simulink model "HOSTFOCwithLOAD"  (R2024b)
settings: Solver=FixedStepDiscrete  StartTime=0.0  StopTime=inf  RelTol=1e-3  EnableMultiTasking=on
PreLoadFcn:
  | % 打开/运行模型时初始化基工作区变量，避免每次启动都要“更新图”
  | if ~exist('dataType','var')
  |     dataType = 'single';   % Data_Conditioning 变体控制（Float/single，与目标机一致）
  | end
  | if ~exist('Ts','var')
  |     Ts = 5e-05;             % 20 kHz，与目标机一致
  | end
  | if ~exist('CalModeP','var')
  |     CalModeP = Simulink.Parameter(uint16(0));
  |     CalModeP.DataType = 'uint16';
  |     CalModeP.CoderInfo.StorageClass = 'Auto';
  | end
InitFcn:
  | % 打开/运行模型时初始化基工作区变量，避免每次启动都要“更新图”
  | if ~exist('dataType','var')
  |     dataType = 'single';   % Data_Conditioning 变体控制（Float/single，与目标机一致）
  | end
  | if ~exist('Ts','var')
  |     Ts = 5e-05;             % 20 kHz，与目标机一致
  | end
  | if exist('CalModeP','var') && isa(CalModeP,'Simulink.Parameter')
  |     CalModeP.Value = uint16(0);
  | else
  |     CalModeP = Simulink.Parameter(uint16(0));
  |     CalModeP.DataType = 'uint16';
  |     CalModeP.CoderInfo.StorageClass = 'Auto';
  | end
undefined symbols (not defined in the file or in its folder): PU_System_motor1, PU_System_motor2
libraries: instrumentseriallib x6, simulink x3
settings Model: Creator=The MathWorks, Inc.  LastModifiedBy=admin
settings SolverCC: AllowMultiTaskInputOutput=on  AlgebraicLoopSolver=TrustRegion  MaxZcPerStep=1
settings DataIOCC: LimitDataPoints=on  SaveFormat=Array  ReturnWorkspaceOutputs=off
settings OptimizationCC: LifeSpan=1  EfficientTunableParamExpr=on
settings DebuggingCC: UnderspecifiedInitializationDetection=Classic  MergeDetectMultiDrivingBlocksExec=none  SolverPrmCheckMsg=warning  ParameterPrecisionLossMsg=none  UnconnectedInputMsg=warning  UnconnectedOutputMsg=warning  UnconnectedLineMsg=warning  AllowSymbolicDim=off  PregeneratedLibrarySubsystemCodeDiagnostic=none  SFUnexpectedBacktrackingDiag=warning  SFNoUnconditionalDefaultTransitionDiag=warning  SFExecutionAtInitializationDiag=none  ArithmeticOperatorsInVariantConditions=warning
settings HardwareCC: ProdBitPerPointer=32  ProdLargestAtomicFloat=None  ProdIntDivRoundTo=Undefined  ProdEndianess=Unspecified  ProdWordSize=32  ProdHWDeviceType=32-bit Generic
settings ModelReferenceCC: EnableRefExpFcnMdlSchedulingChecks=on  PropagateSignalLabelsOutOfModel=off
settings SFSimCC: SimUseLocalCustomCode=off  MATLABDynamicMemAlloc=off
settings RTWCC: Description=Real-Time Workshop Embedded Coder  SystemTargetFile=ert.tlc  TemplateMakefile=ert_default_tmf  GenerateReport=on  RTWUseLocalCustomCode=off  IncludeHyperlinkInReport=on  LaunchReport=on  GenerateTraceInfo=on  GenerateTraceReport=on  GenerateTraceReportSl=on  GenerateTraceReportSf=on  GenerateTraceReportEml=on  GPUComputeCapability=3.5  DLArmComputeVersion=19.05
settings CodeAppCC: IgnoreCustomStorageClasses=off  StateflowObjectComments=on  InternalIdentifier=Classic
settings ERTTargetCC: MultiwordLength=2048  GenerateSampleERTMain=on  InlinedParameterPlacement=Hierarchical  ERTCustomFileTemplate=example_file_process.tlc  ConvertIfToSwitch=off  SuppressUnreachableDefaultCases=off  DynamicArrayContainerType=coder::array
settings ConfigComp: CovMetricSettings=dw  CovSaveCumulativeToWorkspaceVar=on  CovSaveSingleToWorkspaceVar=on  CovExternalEMLEnable=off  CovSFcnEnable=off

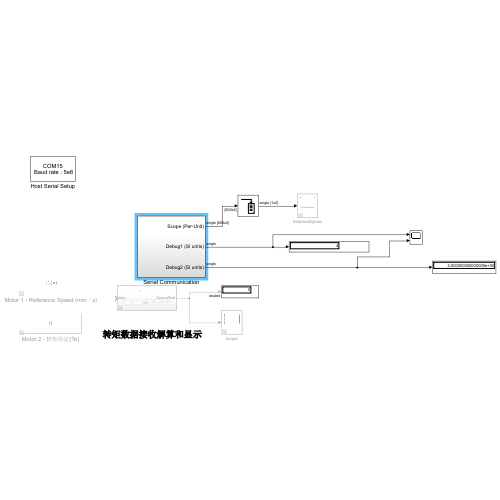
[thumbnail: Simulink's stored preview of the top-level diagram]
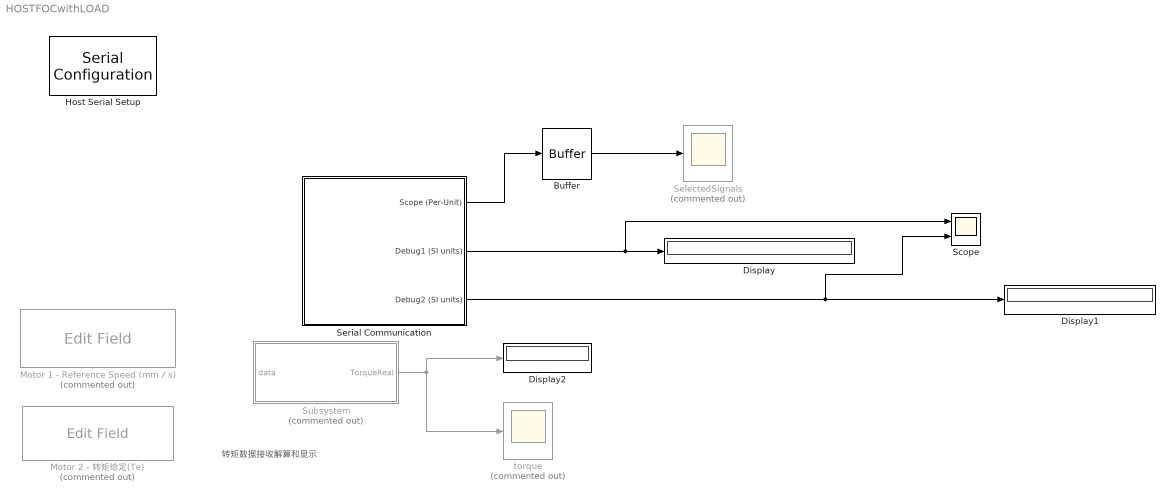
== system HOSTFOCwithLOAD ==
  note: 转矩数据接收解算和显示
  Buffer : Buffer  N=1  OutputFrames=off
  Display : Display
  Display1 : Display
      settings: Format=long_e
  Display2 : Display
  Host Serial Setup : instrumentseriallib/Serial Configuration  Priority=-99  PortSel=COM15  Port=COM15  ComPort=COM15  BaudRate=5e6  DataBits=8  Parity=none  StopBits=1  ByteOrder=little-endian  FlowControl=none  Timeout=2  SimulateUsing=Interpreted execution  BlockInModel=on  aMode=5
  Motor 1 - Reference Speed (mm／s) : EditField  Commented=on  LabelPosition=Hide  ShowInitialText=on  Alignment=Center
  Motor 2 - 转矩给定(Te) : EditField  Commented=on  LabelPosition=Hide  ShowInitialText=on  Alignment=Center
  Scope : Scope  NumInputPorts=2
  SelectedSignals : Scope  Commented=on
  Serial Communication : Subsystem
  Subsystem : Subsystem  Commented=on
  torque : Scope  Commented=on
  wires:
  Serial Communication/2(Debug1 (SI units)) -> Scope/1, Display/1
  Serial Communication/3(Debug2 (SI units)) -> Scope/2, Display1/1
  Serial Communication/1(Scope (Per-Unit)) -> Buffer/1
  Buffer/1 -> SelectedSignals/1
  Subsystem/1(TorqueReal) -> Display2/1, torque/1

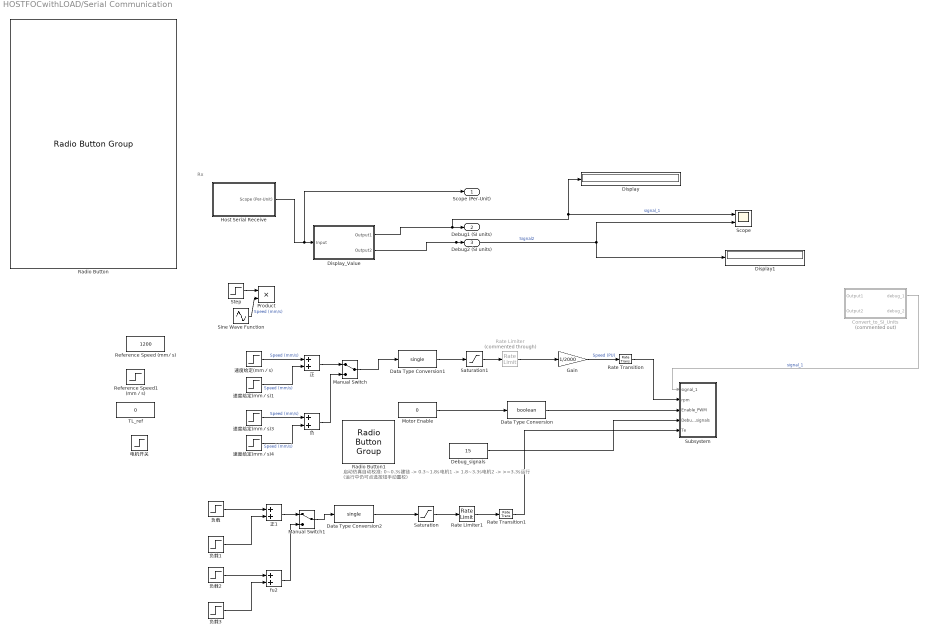
== system HOSTFOCwithLOAD/Serial Communication ==
  note: Rx
  note: 启动仿真自动校准: 0~0.3s建链 -> 0.3~1.8s电机1 -> 1.8~3.3s电机2 -> >=3.3s运行 (运行中仍可点选按钮手动重校)
  Convert_to_SI_Units : Subsystem  Commented=on
  Data Type Conversion : DataTypeConversion  OutDataTypeStr=boolean  SaturateOnIntegerOverflow=off  RndMeth=Floor
  Data Type Conversion1 : DataTypeConversion  OutDataTypeStr=single  SaturateOnIntegerOverflow=off  RndMeth=Floor
  Data Type Conversion2 : DataTypeConversion  OutDataTypeStr=single  SaturateOnIntegerOverflow=off  RndMeth=Floor
  Debug_signals : Constant  Value=15  OutDataTypeStr=uint16  SampleTime=0.03
  Display : Display
  Display1 : Display
      settings: Format=long_e
  Display_Value : MATLAB Function  TreatAsAtomicUnit=on
  Gain : Gain  Gain=1/2000  RndMeth=Simplest  OutDataTypeStr=Inherit: Same as input
  Host Serial Receive : Subsystem  Variant=on
  Manual Switch : ManualSwitch
  Manual Switch1 : ManualSwitch
  Motor Enable : Constant  Value=0  VectorParams1D=off  OutDataTypeStr=uint16  SampleTime=0.03
  Product : Product
  Radio Button : RadioButtonGroup  LabelPosition=Hide  SelectedLabel=iqid_limit  ButtonGroupName=Debug signals
      settings: Values={{'Mtr1: Speed ref & Speed feedback', 'Mtr1: Id ref & Id feedback', 'Mtr1: Iq ref & Iq feedback', 'Mtr1: Vd & Vq', 'Mtr1: Ia & Ib feedback', 'Mtr1: Pm & Te', 'Mtr2: Id ref & Id feedback', 'Mtr2: Iq ref & Iq feedback', 'Mtr2: Vd & Vq', 'Mtr2: Ia & Ib feedback', 'Mtr2: Pm & Te', 'Mtr1&Mtr2: Pm', 'Mtr1&Mtr2: Te', '1&2pos', 'iqid_limit', 'Mtr1 Speed ref & Mtr2 Speed fb'}, [1 2 3 4 5 6 7 8 9 10 11 12 13 14 15 0]}
  Radio Button1 : RadioButtonGroup  SelectedLabel=0 运行  ButtonGroupName=Group
      settings: Values={{'1 校准电机1', '2 校准电机2', '0 运行'}, [1 2 0]}
  Rate Limiter : RateLimiter  Commented=through  RisingSlewLimit=2000  FallingSlewLimit=-2000  SampleTimeMode=inherited
  Rate Limiter1 : RateLimiter  RisingSlewLimit=20  FallingSlewLimit=-20  SampleTimeMode=inherited
  Rate Transition : RateTransition  OutPortSampleTime=0.03
  Rate Transition1 : RateTransition  OutPortSampleTime=0.03
  Reference Speed (mm／s) : Constant  Value=1200  VectorParams1D=off  OutDataTypeStr=single  SampleTime=0
  Reference Speed1 (mm／s) : Step  Time=5  After=1000  OutDataTypeStr=single  SampleTime=0
  Saturation : Saturate  UpperLimit=1  LowerLimit=-1
  Saturation1 : Saturate  UpperLimit=2000  LowerLimit=-2000
  Scope : Scope  NumInputPorts=2
  Sine Wave Function : Sin  Amplitude=250  Frequency=4  SampleTime=0
  Step : Step  Time=7  SampleTime=0
  Subsystem : Subsystem
  TL_ref : Constant  Value=0  VectorParams1D=off  OutDataTypeStr=single  SampleTime=0.03
  fu2 : Sum
  正 : Sum
  正1 : Sum
  电机开关 : Step  Time=400  Before=1  After=0  SampleTime=0.03
  负 : Sum
  负载 : Step  Time=9  After=0.2  OutDataTypeStr=single
  负载1 : Step  Time=10  After=-0.2  OutDataTypeStr=single
  负载2 : Step  Time=9  After=-0.2  OutDataTypeStr=single
  负载3 : Step  Time=10  After=0.2  OutDataTypeStr=single
  速度给定(mm／s) : Step  Time=7  After=250  OutDataTypeStr=single
  速度给定(mm／s)1 : Step  Time=11  After=-250  OutDataTypeStr=single
  速度给定(mm／s)3 : Step  Time=7  After=-250  OutDataTypeStr=single
  速度给定(mm／s)4 : Step  Time=10  After=250  OutDataTypeStr=single
  Scope (Per-Unit) : Outport
  Debug1 (SI units) : Outport  Port=2
  Debug2 (SI units) : Outport  Port=3
  wires:
  Gain/1 -> Rate Transition/1  "Speed (PU)"
  Display_Value/1(Output1) -> Debug1 (SI units)/1, Display/1, Scope/1  "signal_1"
  Display_Value/2(Output2) -> Display1/1, Scope/2, Debug2 (SI units)/1  "Signal2"
  Host Serial Receive/1(Scope (Per-Unit)) -> Display_Value/1(Input), Scope (Per-Unit)/1
  Rate Limiter1/1 -> Rate Transition1/1
  Motor Enable/1 -> Data Type Conversion/1
  Saturation/1 -> Rate Limiter1/1
  Saturation1/1 -> Rate Limiter/1
  Rate Limiter/1 -> Gain/1
  Data Type Conversion1/1 -> Saturation1/1
  Data Type Conversion2/1 -> Saturation/1
  Step/1 -> Product/1
  Sine Wave Function/1 -> Product/2  "Speed (mm/s)"
  Convert_to_SI_Units/1(debug_1) -> Subsystem/1(signal_1)  "signal_1"
  Rate Transition/1 -> Subsystem/2(rpm)
  Data Type Conversion/1 -> Subsystem/3(Enable_PWM)
  Debug_signals/1 -> Subsystem/4(Debug_signals)
  Rate Transition1/1 -> Subsystem/5(Te)
  速度给定(mm／s)/1 -> 正/1  "Speed (mm/s)"
  速度给定(mm／s)1/1 -> 正/2  "Speed (mm/s)"
  正/1 -> Manual Switch/1
  Manual Switch/1 -> Data Type Conversion1/1
  速度给定(mm／s)4/1 -> 负/2  "Speed (mm/s)"
  速度给定(mm／s)3/1 -> 负/1  "Speed (mm/s)"
  负/1 -> Manual Switch/2
  负载1/1 -> 正1/2
  负载/1 -> 正1/1
  正1/1 -> Manual Switch1/1
  Manual Switch1/1 -> Data Type Conversion2/1
  负载3/1 -> fu2/2
  负载2/1 -> fu2/1
  fu2/1 -> Manual Switch1/2

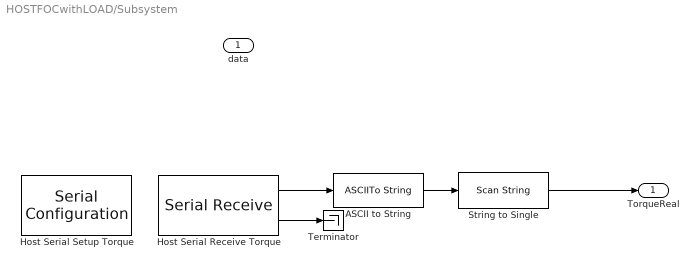
== system HOSTFOCwithLOAD/Subsystem ==
  data : Inport
  ASCII to String : ASCIIToString
  Host Serial Receive Torque : instrumentseriallib/Serial Receive  PortSel=COM7  Port=COM7  ComPort=COM7  DataType=uint8  SaveDataType=uint8  ToggleHeader=off  Header='S'  ToggleDataSize=on  DataSize=[1 7]  ToggleTerminator=on  Terminator=Custom terminator  CustomTerminator=13  InputFormat=Column major  EnableBlockingMode=off  ActionDataUnavailable=Output last received value  ActionWhenDataUnavailable=Output last received value  CustomValue=0  SampleTime=0.001  SimulateUsing=Interpreted execution  BlockInModel=on  aMode=5
      settings: LibrarySourceBlock=mcblib/Protection and Diagnostics/Host Serial Receive
  Host Serial Setup Torque : instrumentseriallib/Serial Configuration  Priority=-99  PortSel=COM7  Port=COM7  ComPort=COM7  BaudRate=19200  DataBits=8  Parity=none  StopBits=1  ByteOrder=little-endian  FlowControl=none  Timeout=2  SimulateUsing=Interpreted execution  BlockInModel=on  aMode=5
  String to Single : ScanString  Format="\"%f\""
  Terminator : Terminator
  TorqueReal : Outport
  wires:
  Host Serial Receive Torque/1 -> ASCII to String/1
  ASCII to String/1 -> String to Single/1
  Host Serial Receive Torque/2 -> Terminator/1
  String to Single/1 -> TorqueReal/1

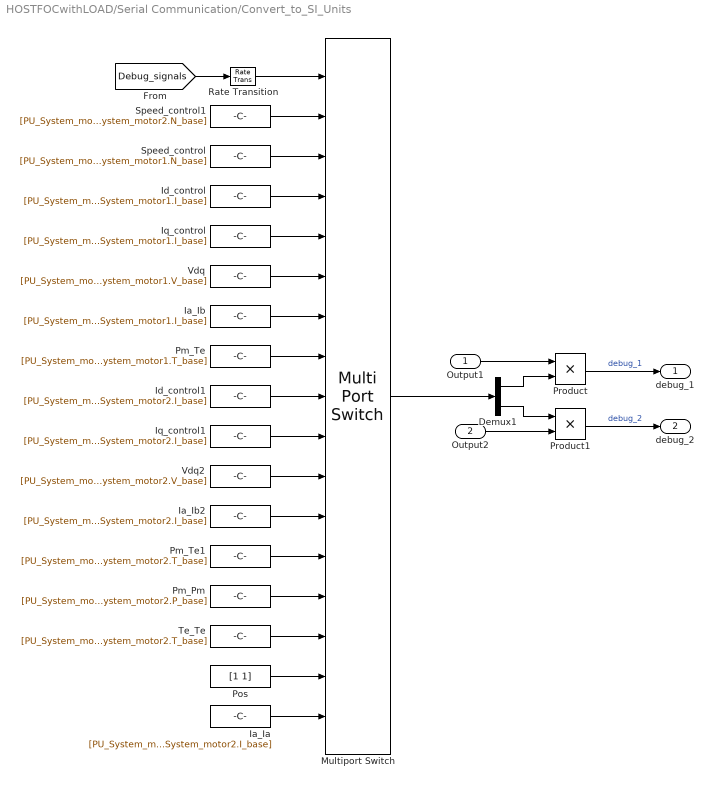
== system HOSTFOCwithLOAD/Serial Communication/Convert_to_SI_Units ==
  Output1 : Inport
  Output2 : Inport  Port=2
  Demux1 : Demux  Outputs=2
  Ia_Ia : Constant  Value=[PU_System_motor1.I_base PU_System_motor2.I_base]  OutDataTypeStr=single  SampleTime=-1
  Ia_Ib : Constant  Value=[PU_System_motor1.I_base PU_System_motor1.I_base]  OutDataTypeStr=single  SampleTime=-1
  Ia_Ib2 : Constant  Value=[PU_System_motor2.I_base PU_System_motor2.I_base]  OutDataTypeStr=single  SampleTime=-1
  Id_control : Constant  Value=[PU_System_motor1.I_base PU_System_motor1.I_base]  OutDataTypeStr=single  SampleTime=-1
  Id_control1 : Constant  Value=[PU_System_motor2.I_base PU_System_motor2.I_base]  OutDataTypeStr=single  SampleTime=-1
  Iq_control : Constant  Value=[PU_System_motor1.I_base PU_System_motor1.I_base]  OutDataTypeStr=single  SampleTime=-1
  Iq_control1 : Constant  Value=[PU_System_motor2.I_base PU_System_motor2.I_base]  OutDataTypeStr=single  SampleTime=-1
  Multiport Switch : MultiPortSwitch  DataPortOrder=Zero-based contiguous  Inputs=16  DiagnosticForDefault=Warning  zeroidx=on  OutDataTypeStr=single  RndMeth=Simplest  SaturateOnIntegerOverflow=off  InputSameDT=off
  Pm_Pm : Constant  Value="[PU_System_motor1.P_base  PU_System_motor2.P_base]"  OutDataTypeStr=single  SampleTime=-1
  Pm_Te : Constant  Value="[PU_System_motor1.P_base  PU_System_motor1.T_base]"  OutDataTypeStr=single  SampleTime=-1
  Pm_Te1 : Constant  Value="[PU_System_motor2.P_base  PU_System_motor2.T_base]"  OutDataTypeStr=single  SampleTime=-1
  Pos : Constant  Value=[1 1]  OutDataTypeStr=single  SampleTime=-1
  Product : Product
  Product1 : Product
  Rate Transition : RateTransition  Deterministic=off
  Speed_control : Constant  Value=[PU_System_motor1.N_base PU_System_motor1.N_base]  OutDataTypeStr=single  SampleTime=-1
  Speed_control1 : Constant  Value=[PU_System_motor1.N_base PU_System_motor2.N_base]  OutDataTypeStr=single  SampleTime=-1
  Te_Te : Constant  Value="[PU_System_motor1.T_base  PU_System_motor2.T_base]"  OutDataTypeStr=single  SampleTime=-1
  Vdq : Constant  Value=[PU_System_motor1.V_base PU_System_motor1.V_base]  OutDataTypeStr=single  SampleTime=-1
  Vdq2 : Constant  Value=[PU_System_motor2.V_base PU_System_motor2.V_base]  OutDataTypeStr=single  SampleTime=-1
  debug_1 : Outport
  debug_2 : Outport  Port=2
  wires:
  Product/1 -> debug_1/1  "debug_1"
  Product1/1 -> debug_2/1  "debug_2"
  [Debug_signals] -> Rate Transition/1
  Multiport Switch/1 -> Demux1/1
  Demux1/1 -> Product/2
  Output1/1 -> Product/1
  Rate Transition/1 -> Multiport Switch/1
  Pos/1 -> Multiport Switch/16
  Ia_Ia/1 -> Multiport Switch/17
  Te_Te/1 -> Multiport Switch/15
  Pm_Pm/1 -> Multiport Switch/14
  Pm_Te1/1 -> Multiport Switch/13
  Ia_Ib2/1 -> Multiport Switch/12
  Vdq2/1 -> Multiport Switch/11
  Iq_control1/1 -> Multiport Switch/10
  Id_control1/1 -> Multiport Switch/9
  Pm_Te/1 -> Multiport Switch/8
  Ia_Ib/1 -> Multiport Switch/7
  Vdq/1 -> Multiport Switch/6
  Iq_control/1 -> Multiport Switch/5
  Id_control/1 -> Multiport Switch/4
  Speed_control/1 -> Multiport Switch/3
  Speed_control1/1 -> Multiport Switch/2
  Demux1/2 -> Product1/1
  Output2/1 -> Product1/2

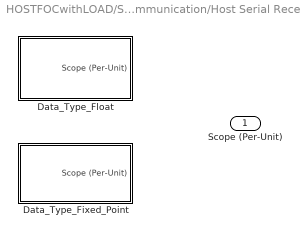
== system HOSTFOCwithLOAD/Serial Communication/Host Serial Receive ==
  Data_Type_Fixed_Point : Subsystem  VariantControl=~isequal(dataType, 'single')
  Data_Type_Float : Subsystem  VariantControl=isequal(dataType, 'single')
  Scope (Per-Unit) : Outport

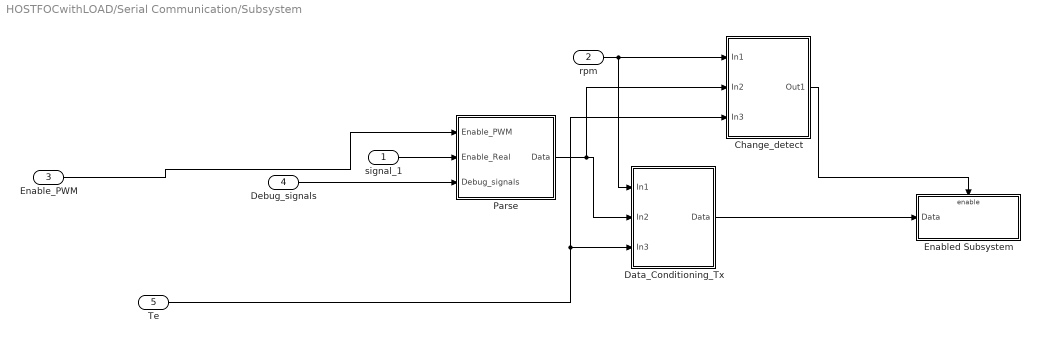
== system HOSTFOCwithLOAD/Serial Communication/Subsystem ==
  signal_1 : Inport
  rpm : Inport  Port=2
  Enable_PWM : Inport  Port=3
  Debug_signals : Inport  Port=4
  Te : Inport  Port=5
  Change_detect : Subsystem
  Data_Conditioning_Tx : Subsystem  Variant=on
  Enabled Subsystem : Subsystem  TreatAsAtomicUnit=on
  Parse : Subsystem
  wires:
  Enable_PWM/1 -> Parse/1(Enable_PWM)
  Parse/1(Data) -> Data_Conditioning_Tx/2(In2), Change_detect/2(In2)
  rpm/1 -> Change_detect/1(In1), Data_Conditioning_Tx/1(In1)
  signal_1/1 -> Parse/2(Enable_Real)
  Te/1 -> Data_Conditioning_Tx/3(In3), Change_detect/3(In3)
  Change_detect/1(Out1) -> Enabled Subsystem/Enable
  Data_Conditioning_Tx/1(Data) -> Enabled Subsystem/1(Data)
  Debug_signals/1 -> Parse/3(Debug_signals)

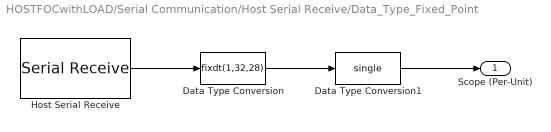
== system HOSTFOCwithLOAD/Serial Communication/Host Serial Receive/Data_Type_Fixed_Point ==
  Data Type Conversion : DataTypeConversion  OutDataTypeStr=fixdt(1,32,28)  ConvertRealWorld=Stored Integer (SI)  RndMeth=Simplest  SaturateOnIntegerOverflow=off
  Data Type Conversion1 : DataTypeConversion  OutDataTypeStr=single  RndMeth=Simplest  SaturateOnIntegerOverflow=off
  Host Serial Receive : instrumentseriallib/Serial Receive  PortSel=<Select a port...>  Port=<Select a port...>  ComPort=<Select a port...>  DataType=uint32  SaveDataType=uint8  ToggleHeader=on  Header='SSSS'  ToggleDataSize=on  DataSize=[600 2]  ToggleTerminator=on  Terminator=Custom terminator  CustomTerminator='EEEE'  InputFormat=Row major  EnableBlockingMode=on  ActionDataUnavailable=Output custom value  ActionWhenDataUnavailable=Output custom value  CustomValue=4  SampleTime=600*Ts  SimulateUsing=Interpreted execution  BlockInModel=on  aMode=5
  Scope (Per-Unit) : Outport
  wires:
  Data Type Conversion/1 -> Data Type Conversion1/1
  Host Serial Receive/1 -> Data Type Conversion/1
  Data Type Conversion1/1 -> Scope (Per-Unit)/1

== system HOSTFOCwithLOAD/Serial Communication/Host Serial Receive/Data_Type_Float ==
  Host Serial Receive : instrumentseriallib/Serial Receive  PortSel=target.comport  Port=target.comport  ComPort=target.comport  DataType=single  SaveDataType=uint8  ToggleHeader=on  Header='SSSS'  ToggleDataSize=on  DataSize=[600 2]  ToggleTerminator=on  Terminator=Custom terminator  CustomTerminator='EEEE'  InputFormat=Row major  EnableBlockingMode=on  ActionDataUnavailable=Output custom value  ActionWhenDataUnavailable=Output custom value  CustomValue=4  SampleTime=600*Ts  SimulateUsing=Interpreted execution  BlockInModel=on  aMode=5
  Scope (Per-Unit) : Outport
  wires:
  Host Serial Receive/1 -> Scope (Per-Unit)/1

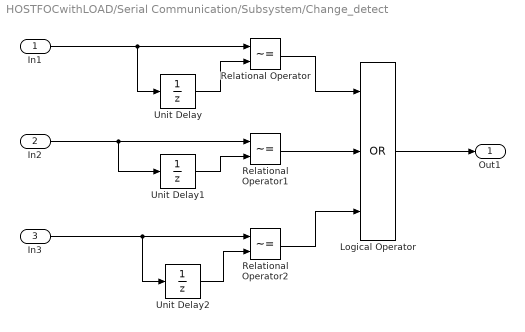
== system HOSTFOCwithLOAD/Serial Communication/Subsystem/Change_detect ==
  In1 : Inport
  In2 : Inport  Port=2
  In3 : Inport  Port=3
  Logical Operator : Logic  Operator=OR  Inputs=3  AllPortsSameDT=off  OutDataTypeStr=boolean
  Relational Operator : RelationalOperator  Operator=~=  OutDataTypeStr=boolean  InputSameDT=off
  Relational Operator1 : RelationalOperator  Operator=~=  OutDataTypeStr=boolean  InputSameDT=off
  Relational Operator2 : RelationalOperator  Operator=~=  OutDataTypeStr=boolean  InputSameDT=off
  Unit Delay : UnitDelay  InitialCondition=0.5  SampleTime=-1  HasFrameUpgradeWarning=on
  Unit Delay1 : UnitDelay  SampleTime=-1  HasFrameUpgradeWarning=on
  Unit Delay2 : UnitDelay  InitialCondition=0.5  SampleTime=-1  HasFrameUpgradeWarning=on
  Out1 : Outport  VectorParamsAs1DForOutWhenUnconnected=off
  wires:
  In2/1 -> Relational Operator1/1, Unit Delay1/1
  Relational Operator1/1 -> Logical Operator/2
  Unit Delay1/1 -> Relational Operator1/2
  Unit Delay/1 -> Relational Operator/2
  In1/1 -> Unit Delay/1, Relational Operator/1
  Relational Operator/1 -> Logical Operator/1
  Logical Operator/1 -> Out1/1
  Relational Operator2/1 -> Logical Operator/3
  Unit Delay2/1 -> Relational Operator2/2
  In3/1 -> Unit Delay2/1, Relational Operator2/1

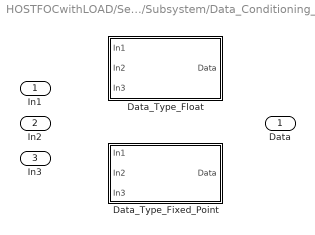
== system HOSTFOCwithLOAD/Serial Communication/Subsystem/Data_Conditioning_Tx ==
  In1 : Inport
  In2 : Inport  Port=2
  In3 : Inport  Port=3
  Data_Type_Fixed_Point : Subsystem  VariantControl=~isequal(dataType, 'single')
  Data_Type_Float : Subsystem  VariantControl=isequal(dataType, 'single')
  Data : Outport

== system HOSTFOCwithLOAD/Serial Communication/Subsystem/Enabled Subsystem ==
  Data : Inport
  Enable : EnablePort
  Host Serial Transmit : instrumentseriallib/Serial Send  PortSel=target.comport  Port=target.comport  ComPort=target.comport  Header=[170 85]  Terminator=Custom terminator  CustomTerminator=[85 170]  EnableBlockingMode=off  SimulateUsing=Interpreted execution  BlockInModel=on  aMode=5
  wires:
  Data/1 -> Host Serial Transmit/1

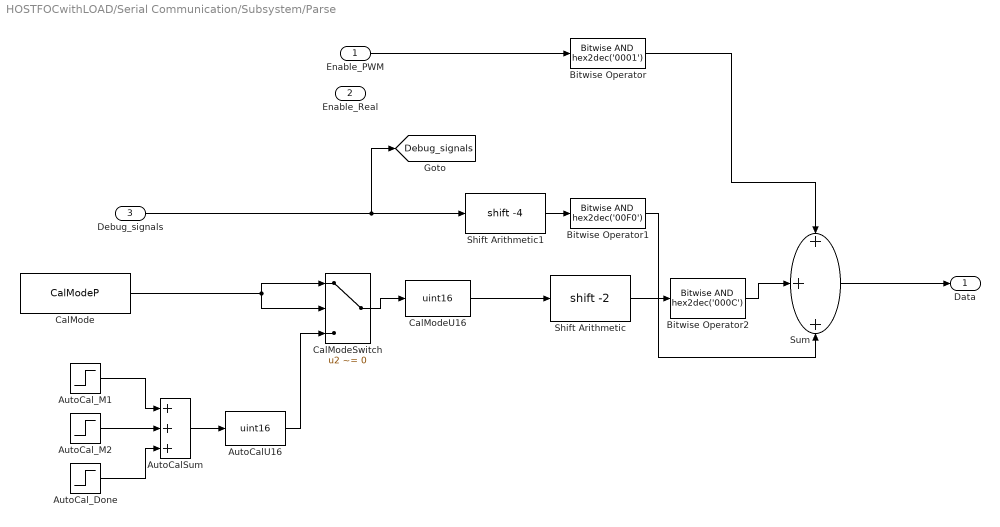
== system HOSTFOCwithLOAD/Serial Communication/Subsystem/Parse ==
  Enable_PWM : Inport
  Enable_Real : Inport  Port=2
  Debug_signals : Inport  Port=3
  AutoCalSum : Sum  Inputs=+++
  AutoCalU16 : DataTypeConversion  OutDataTypeStr=uint16  RndMeth=Floor
  AutoCal_Done : Step  Time=3.3 - 1e-6  After=-2  SampleTime=0.03
  AutoCal_M1 : Step  Time=0.3 - 1e-6  SampleTime=0.03
  AutoCal_M2 : Step  Time=1.8 - 1e-6  SampleTime=0.03
  Bitwise Operator : simulink/Logic and Bit Operations/Bitwise Operator  logicop=AND  UseBitMask=on  BitMask=hex2dec('0001')  BitMaskRealWorld=Stored Integer
  Bitwise Operator1 : simulink/Logic and Bit Operations/Bitwise Operator  logicop=AND  UseBitMask=on  BitMask=hex2dec('00F0')  BitMaskRealWorld=Stored Integer
  Bitwise Operator2 : simulink/Logic and Bit Operations/Bitwise Operator  logicop=AND  UseBitMask=on  BitMask=hex2dec('000C')  BitMaskRealWorld=Stored Integer
  CalMode : Constant  Value=CalModeP  OutDataTypeStr=uint16
  CalModeSwitch : Switch  Criteria=u2 ~= 0  OutDataTypeStr=uint16  SaturateOnIntegerOverflow=off  InputSameDT=off
  CalModeU16 : DataTypeConversion  OutDataTypeStr=uint16
  Shift Arithmetic1 : ArithShift  BitShiftNumber=-4
  Shift Arithmetic : ArithShift  BitShiftNumber=-2
  Sum : Sum  Inputs=+++
  Data : Outport
  tag scope: Debug_signals=global
  wires:
  Debug_signals/1 -> Shift Arithmetic1/1, [Debug_signals]
  Shift Arithmetic1/1 -> Bitwise Operator1/1
  Enable_PWM/1 -> Bitwise Operator/1
  Shift Arithmetic/1 -> Bitwise Operator2/1
  Bitwise Operator2/1 -> Sum/2
  Sum/1 -> Data/1
  CalModeU16/1 -> Shift Arithmetic/1
  Bitwise Operator/1 -> Sum/1
  Bitwise Operator1/1 -> Sum/3
  AutoCal_M1/1 -> AutoCalSum/1
  AutoCal_M2/1 -> AutoCalSum/2
  AutoCal_Done/1 -> AutoCalSum/3
  AutoCalSum/1 -> AutoCalU16/1
  CalMode/1 -> CalModeSwitch/1, CalModeSwitch/2
  AutoCalU16/1 -> CalModeSwitch/3
  CalModeSwitch/1 -> CalModeU16/1

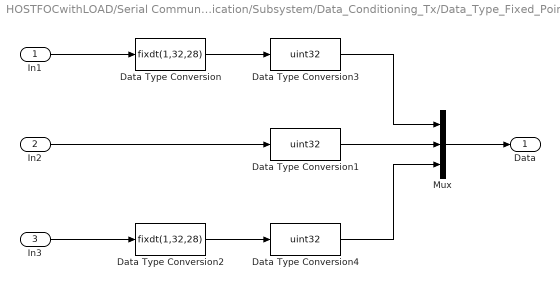
== system HOSTFOCwithLOAD/Serial Communication/Subsystem/Data_Conditioning_Tx/Data_Type_Fixed_Point ==
  In1 : Inport
  In2 : Inport  Port=2
  In3 : Inport  Port=3
  Data Type Conversion : DataTypeConversion  OutDataTypeStr=fixdt(1,32,28)  RndMeth=Simplest  SaturateOnIntegerOverflow=off
  Data Type Conversion1 : DataTypeConversion  OutDataTypeStr=uint32  RndMeth=Simplest  SaturateOnIntegerOverflow=off
  Data Type Conversion2 : DataTypeConversion  OutDataTypeStr=fixdt(1,32,28)  RndMeth=Simplest  SaturateOnIntegerOverflow=off
  Data Type Conversion3 : DataTypeConversion  OutDataTypeStr=uint32  ConvertRealWorld=Stored Integer (SI)  RndMeth=Simplest  SaturateOnIntegerOverflow=off
  Data Type Conversion4 : DataTypeConversion  OutDataTypeStr=uint32  ConvertRealWorld=Stored Integer (SI)  RndMeth=Simplest  SaturateOnIntegerOverflow=off
  Mux : Mux  Inputs=3
  Data : Outport
  wires:
  In1/1 -> Data Type Conversion/1
  Data Type Conversion3/1 -> Mux/1
  Data Type Conversion/1 -> Data Type Conversion3/1
  In2/1 -> Data Type Conversion1/1
  Data Type Conversion1/1 -> Mux/2
  Mux/1 -> Data/1
  Data Type Conversion2/1 -> Data Type Conversion4/1
  Data Type Conversion4/1 -> Mux/3
  In3/1 -> Data Type Conversion2/1

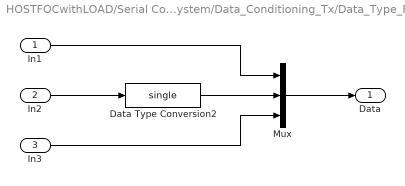
== system HOSTFOCwithLOAD/Serial Communication/Subsystem/Data_Conditioning_Tx/Data_Type_Float ==
  In1 : Inport
  In2 : Inport  Port=2
  In3 : Inport  Port=3
  Data Type Conversion2 : DataTypeConversion  OutDataTypeStr=single  RndMeth=Simplest  SaturateOnIntegerOverflow=off
  Mux : Mux  Inputs=3
  Data : Outport
  wires:
  In1/1 -> Mux/1
  Mux/1 -> Data/1
  In2/1 -> Data Type Conversion2/1
  Data Type Conversion2/1 -> Mux/2
  In3/1 -> Mux/3

== matlab function HOSTFOCwithLOAD/Serial Communication/Display_Value ==
  data: Output1 output; Input input; Output2 output
function [Output1, Output2] = unBuf (Input)
%% ************************************************************************
% Unbuffer function
% Outputs first received serial data from buffer for both signals

% Copyright 2020 The MathWorks, Inc.

selSignal= Input(:, 1);
Output1 = selSignal(1,1);
selSignal = Input(:, 2);
Output2 = selSignal(1,1);
end
